simulink model "HERIC"  (R2025a)
settings: Solver=VariableStepAuto  StartTime=0.0  StopTime=1  RelTol=1e-3
libraries: spsMosfetLib x8, spsSeriesRLCBranchLib x7, spsDiodeLib x2, simulink x2, spsDCVoltageSourceLib x1, spspowerguiLib x1
settings Model: Creator=Mohamed Ibrahim  LastModifiedBy=Mohamed Ibrahim

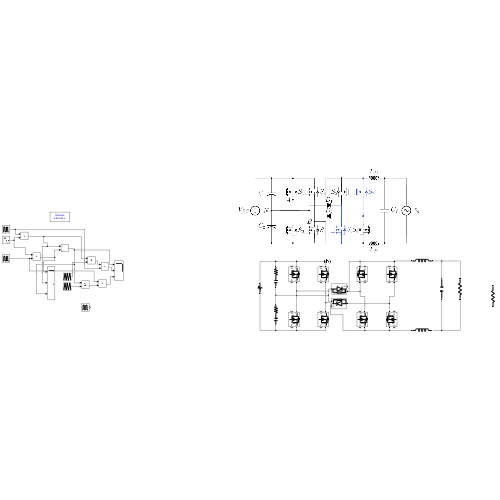
[thumbnail: Simulink's stored preview of the top-level diagram]
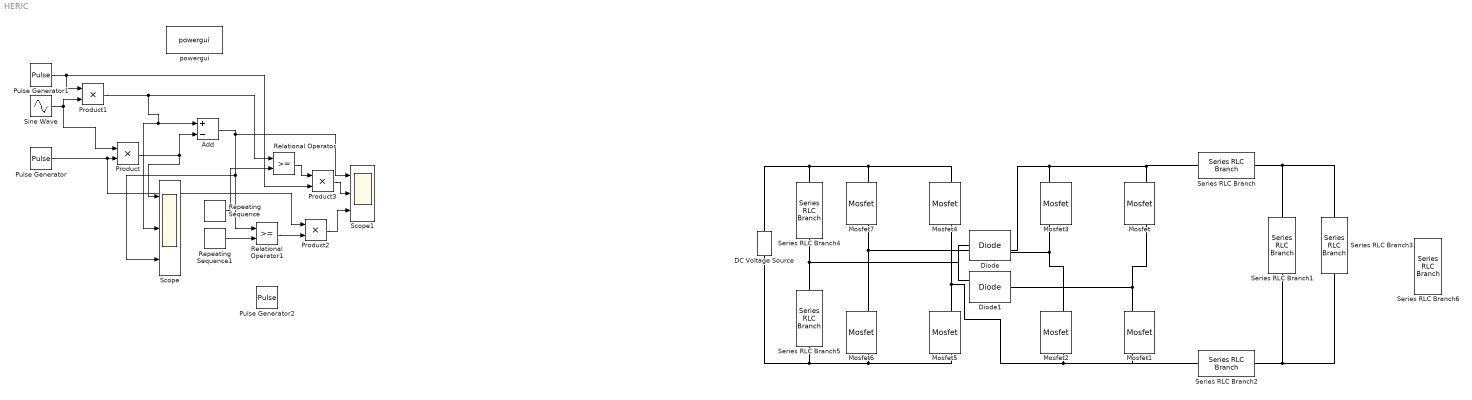
== system HERIC ==
  Add : Sum  Inputs=+-
  DC Voltage Source : spsDCVoltageSourceLib/DC Voltage Source  Amplitude=100  Measurements=None
  Diode : spsDiodeLib/Diode  Ron=0.001  Lon=0  Vf=0.8  IC=0  UseSnubber=0  Rs=500  Cs=250e-9  Measurements=on
  Diode1 : spsDiodeLib/Diode  Ron=0.001  Lon=0  Vf=0.8  IC=0  UseSnubber=0  Rs=500  Cs=250e-9  Measurements=on
  Mosfet{,1..7} (8 alike) : spsMosfetLib/Mosfet  Ron=0.1  Lon=0  Rd=0.01  Vfd=0  IC=0  Rs=1e5  Cs=inf  Measurements=on
  Product{,1..3} (4 alike) : Product
  Pulse Generator : DiscretePulseGenerator  PulseType=Time based  Period=0.02  PulseWidth=50  PhaseDelay=0.01
  Pulse Generator1 : DiscretePulseGenerator  PulseType=Time based  Period=0.02  PulseWidth=50
  Pulse Generator2 : DiscretePulseGenerator  PulseType=Time based  Period=0.02  PulseWidth=50  PhaseDelay=0.01
  Relational Operator : RelationalOperator  OutDataTypeStr=boolean  RndMeth=Simplest  InputSameDT=off
  Relational Operator1 : RelationalOperator  OutDataTypeStr=boolean  RndMeth=Simplest  InputSameDT=off
  Repeating Sequence : simulink/Sources/Repeating Sequence  rep_seq_t=[0 0.000025 0.00005]  rep_seq_y=[0 1 0]
  Repeating Sequence1 : simulink/Sources/Repeating Sequence  rep_seq_t=[0.000025 0.00005 0.000075]  rep_seq_y=[0 1 0]
  Scope : Scope  NumInputPorts=3
      settings: ActiveDisplayYMinimum=-1  ActiveDisplayYMaximum=1
  Scope1 : Scope  NumInputPorts=3
      settings: ActiveDisplayYMinimum=-0.12500000000002531  ActiveDisplayYMaximum=1.1250000000000029
  Series RLC Branch : spsSeriesRLCBranchLib/Series RLC Branch  LConnTagsString=__new0  RConnTagsString=__new0  BranchType=L  Resistance=1  Inductance=1e-3  SetiL0=off  InitialCurrent=0  Capacitance=1e-6  Setx0=off  InitialVoltage=0  Measurements=None
  Series RLC Branch1 : spsSeriesRLCBranchLib/Series RLC Branch  LConnTagsString=__new0  RConnTagsString=__new0  BranchType=C  Resistance=1  Inductance=1e-3  SetiL0=off  InitialCurrent=0  Capacitance=1e-6  Setx0=off  InitialVoltage=0  Measurements=None
  Series RLC Branch2 : spsSeriesRLCBranchLib/Series RLC Branch  LConnTagsString=__new0  RConnTagsString=__new0  BranchType=L  Resistance=1  Inductance=1e-3  SetiL0=off  InitialCurrent=0  Capacitance=1e-6  Setx0=off  InitialVoltage=0  Measurements=None
  Series RLC Branch3 : spsSeriesRLCBranchLib/Series RLC Branch  LConnTagsString=__new0  RConnTagsString=__new0  BranchType=R  Resistance=1  Inductance=1e-3  SetiL0=off  InitialCurrent=0  Capacitance=1e-6  Setx0=off  InitialVoltage=0  Measurements=None
  Series RLC Branch4 : spsSeriesRLCBranchLib/Series RLC Branch  LConnTagsString=__new0  RConnTagsString=__new0  BranchType=RC  Resistance=1  Inductance=1e-3  SetiL0=off  InitialCurrent=0  Capacitance=1e-6  Setx0=off  InitialVoltage=0  Measurements=None
  Series RLC Branch5 : spsSeriesRLCBranchLib/Series RLC Branch  LConnTagsString=__new0  RConnTagsString=__new0  BranchType=RC  Resistance=1  Inductance=1e-3  SetiL0=off  InitialCurrent=0  Capacitance=1e-6  Setx0=off  InitialVoltage=0  Measurements=None
  Series RLC Branch6 : spsSeriesRLCBranchLib/Series RLC Branch  LConnTagsString=__new0  RConnTagsString=__new0  BranchType=R  Resistance=1  Inductance=1e-3  SetiL0=off  InitialCurrent=0  Capacitance=1e-6  Setx0=off  InitialVoltage=0  Measurements=None
  Sine Wave : Sin  Frequency=2*pi*50  SampleTime=0
  powergui : spspowerguiLib/powergui  Priority=1  SimulationMode=Discrete  SampleTime=6.25e-6  frequency=60  Iterations=50  frequencyindice=0  Pbase=100e6  ErrMax=1e-4  UnitsV=kV  UnitsW=MW  buscounter=0  FunctionMessages=off  echomessages=off  EnableUseOfTLC=off  CurrentSourceSwitches=off  DisableSnubberDevices=off  DisableRonSwitches=off  DisableVfSwitches=off  DisplayEquations=off  AutomaticDiscreteSolvers=off  SolverType=Tustin/Backward Euler (TBE)  Interpol=off  ExternalGateDelay=off  methode=off  Ts=100  x0status=blocks  SPID=on  SwTol=0  HookPort=off  NonlinearTolerance=1e-4  nMaxIteration=100  ContinueOnMaxIteration=off  RestoreLinks=warning  ResistiveCurrentMeasurement=off  Frange=[0:2:500]  Ylog=off  Xlog=on  ShowGrid=off  save=off  variable=ZData  structure=0  ZoomFFT=off  StartTime=0.0  cycles=1  DisplayStyle=1  fundamental=60  FreqAxis=off  MaxFrequency=1000  frequencyindicesteady=1  RmsSteady=1  display=off
  wires:
  Pulse Generator/1 -> Product2/1, Product/2
  Product1/1 -> Relational Operator/1, Add/1, Scope/2
  Product/1 -> Add/2, Scope/1
  Add/1 -> Scope1/1, Relational Operator1/1, Scope/3
  Sine Wave/1 -> Product/1, Product1/2
  Pulse Generator1/1 -> Product3/2, Product1/1
  Repeating Sequence/1 -> Relational Operator/2
  Repeating Sequence1/1 -> Relational Operator1/2
  Relational Operator1/1 -> Product2/2
  Product2/1 -> Scope1/3
  Product3/1 -> Scope1/2
  Relational Operator/1 -> Product3/1
  connections:
  DC Voltage Source/RConn1 -- Series RLC Branch4/LConn1 -- Mosfet4/LConn1 -- Mosfet7/LConn1
  Mosfet2/LConn1 -- Mosfet3/LConn1 -- Diode/RConn1
  Mosfet1/RConn1 -- Mosfet/RConn1 -- Diode1/LConn1
  Mosfet5/LConn1 -- Series RLC Branch2/LConn1 -- Mosfet1/LConn1 -- Mosfet2/RConn1 -- Mosfet4/RConn1
  Series RLC Branch5/LConn1 -- Diode/LConn1 -- Diode1/RConn1 -- Series RLC Branch4/RConn1
  Series RLC Branch1/LConn1 -- Series RLC Branch3/LConn1 -- Series RLC Branch/RConn1
  Series RLC Branch2/RConn1 -- Series RLC Branch3/RConn1 -- Series RLC Branch1/RConn1
  Series RLC Branch5/RConn1 -- DC Voltage Source/LConn1 -- Mosfet5/RConn1 -- Mosfet6/RConn1
  Mosfet7/RConn1 -- Mosfet6/LConn1 -- Mosfet/LConn1 -- Series RLC Branch/LConn1 -- Mosfet3/RConn1
